simulink model "s_b2a4x1kf"  (R2018b)
settings: Solver=VariableStepDiscrete  StartTime=0.0  StopTime=100  RelTol=1e-3
undefined symbols (not defined in the file): fft_stages, n_bits_ants, n_bits_xengs
libraries: xbsIndex_r4 x20671, casper_library_misc x69, casper_library_scopes x15, casper_library_delays x8, xbsReplacements_r4 x6, xps_library x4
(part 152 of 212)

== system s_b2a4x1kf/sys0/xeng/baseline_tap1/dual_pol_cmac/cmac1 ==
  a+bi : Inport
  c+di : Inport  Port=2
  acc_in : Inport  Port=3
  sync : Inport  Port=4
  valid_in : Inport  Port=5
  Constant1 : xbsIndex_r4/Constant  const=0  gui_display_data_type=Fixed-point  arith_type=Unsigned  n_bits=bit_growth  bin_pt=0  preci_type=Single  exp_width=8  frac_width=24  explicit_period=on  period=1  equ=P=C  opselect=C  inp2=PCIN>>17  opr=+  inp1=P  carry=CIN  dbl_ovrd=off  block_type=constant
      settings: block_version=9.2.01
  Constant2 : xbsIndex_r4/Constant  const=0  gui_display_data_type=Fixed-point  arith_type=Unsigned  n_bits=1  bin_pt=0  preci_type=Single  exp_width=8  frac_width=24  explicit_period=off  period=1  equ=P=C  opselect=C  inp2=PCIN>>17  opr=+  inp1=P  carry=CIN  dbl_ovrd=off  block_type=constant
      settings: block_version=9.2.01
  Counter : xbsIndex_r4/Counter  cnt_type=Count Limited  cnt_to=acc_len - 1  operation=Up  start_count=0  cnt_by_val=1  arith_type=Unsigned  n_bits=bit_growth  bin_pt=0  load_pin=off  rst=on  en=off  explicit_period=off  period=1  use_behavioral_HDL=off  implementation=Fabric  use_rpm=on  dbl_ovrd=off  block_type=counter
      settings: xl_area=[0, 0, 0, 0, 0, 0, 0]  block_version=9.2.01
  Delay : xbsIndex_r4/Delay  rst=off  infoeditControl=Selection of Reset will increase slice count due to use of real FFs and instead of SRLs  en=off  latency=add_latency + mult_latency - 1  reg_retiming=on  dbl_ovrd=off  block_type=delay
      settings: xl_area=[0, 0, 0, 0, 0, 0, 0]  block_version=9.2.01
  Relational : xbsIndex_r4/Relational  mode=a=b  op_type=Bool  en=off  latency=1  dbl_ovrd=off  block_type=relational
      settings: xl_area=[0, 0, 0, 0, 0, 0, 0]  block_version=9.2.01
  Terminator : Terminator
  acc : Subsystem
  acc1 : Subsystem
  c_to_ri1 : Subsystem
  c_to_ri2 : Subsystem
  cmult* : Subsystem  AncestorBlock=casper_library_multipliers/cmult  mask(cmult){n_bits_a=8, bin_pt_a=7, n_bits_b=8, bin_pt_b=7, n_bits_ab=25, bin_pt_ab=14, quantization=Truncate, overflow=Wrap, in_latency=0, mult_latency=4, add_latency=3, conv_latency=0, conjugated=on, async=off, pipelined_enable=on, multiplier_implementation=embedded multiplier core}
      mask prompts: n_bits_a "Number of Bits 'a'"; bin_pt_a "Binary Point 'a'"; n_bits_b "Number of Bits 'b'"; bin_pt_b "Binary Point 'b'"; n_bits_ab "Number of Bits 'ab'"; bin_pt_ab "Binary Point 'ab'"; in_latency "Input latency"; mult_latency "Multiplier Latency"; add_latency "Adder Latency"; conv_latency "Convert latency"; conjugated "Conjugate"; async "asynchronous operation"; pipelined_enable "enable pipeline"; multiplier_implementation "Multiplier implementation"
      mask help:
      | Multiplies two complex numbers using 4 multipliers and 2 adders.
      | Conjugation is optional.
      mask init: same as s_b2a4x1kf/sys0/xeng/auto_tap/dual_pol_cmac/cmac/cmult*
      settings: AttributesFormatString=|
      | 8_7 * 8_7 ==> 25_14
      | Truncate, Wrap
      | Latency=0
      mask TypeOptions quantization: Truncate | Round  (unbiased: +/- Inf) | Round  (unbiased: Even Values)
      mask TypeOptions overflow: Wrap | Saturate | Flag as error
      mask TypeOptions multiplier_implementation: behavioral HDL | standard core | embedded multiplier core
  ri_to_c : Subsystem
  acc_out : Outport
  valid_out : Outport  Port=2
  wires:
  cmult*/1(ab) -> c_to_ri1/1(In1)
  valid_in/1 -> acc1/4(valid_in)
  acc1/2(valid_out) -> valid_out/1
  acc/2(valid_out) -> Terminator/1
  Constant2/1 -> acc/4(valid_in)
  Delay/1 -> Counter/1
  sync/1 -> Delay/1
  Constant1/1 -> Relational/2
  Counter/1 -> Relational/1
  Relational/1 -> acc1/1(rst), acc/1(rst)
  c_to_ri2/2(Out2) -> acc1/3(acc_in)
  ri_to_c/1(Out1) -> acc_out/1
  acc1/1(acc_out) -> ri_to_c/2(In2)
  acc_in/1 -> c_to_ri2/1(In1)
  c+di/1 -> cmult*/2(b)
  a+bi/1 -> cmult*/1(a)
  c_to_ri1/1(Out1) -> acc/2(din)  "auto_real"
  c_to_ri1/2(Out2) -> acc1/2(din)
  acc/1(acc_out) -> ri_to_c/1(In1)
  c_to_ri2/1(Out1) -> acc/3(acc_in)

== system s_b2a4x1kf/sys0/xeng/baseline_tap1/dual_pol_cmac/cmac2 ==
  a+bi : Inport
  c+di : Inport  Port=2
  acc_in : Inport  Port=3
  sync : Inport  Port=4
  valid_in : Inport  Port=5
  Constant1 : xbsIndex_r4/Constant  const=0  gui_display_data_type=Fixed-point  arith_type=Unsigned  n_bits=bit_growth  bin_pt=0  preci_type=Single  exp_width=8  frac_width=24  explicit_period=on  period=1  equ=P=C  opselect=C  inp2=PCIN>>17  opr=+  inp1=P  carry=CIN  dbl_ovrd=off  block_type=constant
      settings: block_version=9.2.01
  Constant2 : xbsIndex_r4/Constant  const=0  gui_display_data_type=Fixed-point  arith_type=Unsigned  n_bits=1  bin_pt=0  preci_type=Single  exp_width=8  frac_width=24  explicit_period=off  period=1  equ=P=C  opselect=C  inp2=PCIN>>17  opr=+  inp1=P  carry=CIN  dbl_ovrd=off  block_type=constant
      settings: block_version=9.2.01
  Counter : xbsIndex_r4/Counter  cnt_type=Count Limited  cnt_to=acc_len - 1  operation=Up  start_count=0  cnt_by_val=1  arith_type=Unsigned  n_bits=bit_growth  bin_pt=0  load_pin=off  rst=on  en=off  explicit_period=off  period=1  use_behavioral_HDL=off  implementation=Fabric  use_rpm=on  dbl_ovrd=off  block_type=counter
      settings: xl_area=[0, 0, 0, 0, 0, 0, 0]  block_version=9.2.01
  Delay : xbsIndex_r4/Delay  rst=off  infoeditControl=Selection of Reset will increase slice count due to use of real FFs and instead of SRLs  en=off  latency=add_latency + mult_latency - 1  reg_retiming=on  dbl_ovrd=off  block_type=delay
      settings: xl_area=[0, 0, 0, 0, 0, 0, 0]  block_version=9.2.01
  Relational : xbsIndex_r4/Relational  mode=a=b  op_type=Bool  en=off  latency=1  dbl_ovrd=off  block_type=relational
      settings: xl_area=[0, 0, 0, 0, 0, 0, 0]  block_version=9.2.01
  Terminator : Terminator
  acc : Subsystem
  acc1 : Subsystem
  c_to_ri1 : Subsystem
  c_to_ri2 : Subsystem
  cmult* : Subsystem  AncestorBlock=casper_library_multipliers/cmult  mask(cmult){n_bits_a=8, bin_pt_a=7, n_bits_b=8, bin_pt_b=7, n_bits_ab=25, bin_pt_ab=14, quantization=Truncate, overflow=Wrap, in_latency=0, mult_latency=4, add_latency=3, conv_latency=0, conjugated=on, async=off, pipelined_enable=on, multiplier_implementation=embedded multiplier core}
      mask prompts: n_bits_a "Number of Bits 'a'"; bin_pt_a "Binary Point 'a'"; n_bits_b "Number of Bits 'b'"; bin_pt_b "Binary Point 'b'"; n_bits_ab "Number of Bits 'ab'"; bin_pt_ab "Binary Point 'ab'"; in_latency "Input latency"; mult_latency "Multiplier Latency"; add_latency "Adder Latency"; conv_latency "Convert latency"; conjugated "Conjugate"; async "asynchronous operation"; pipelined_enable "enable pipeline"; multiplier_implementation "Multiplier implementation"
      mask help:
      | Multiplies two complex numbers using 4 multipliers and 2 adders.
      | Conjugation is optional.
      mask init: same as s_b2a4x1kf/sys0/xeng/auto_tap/dual_pol_cmac/cmac/cmult*
      settings: AttributesFormatString=|
      | 8_7 * 8_7 ==> 25_14
      | Truncate, Wrap
      | Latency=0
      mask TypeOptions quantization: Truncate | Round  (unbiased: +/- Inf) | Round  (unbiased: Even Values)
      mask TypeOptions overflow: Wrap | Saturate | Flag as error
      mask TypeOptions multiplier_implementation: behavioral HDL | standard core | embedded multiplier core
  ri_to_c : Subsystem
  acc_out : Outport
  valid_out : Outport  Port=2
  wires:
  cmult*/1(ab) -> c_to_ri1/1(In1)
  valid_in/1 -> acc1/4(valid_in)
  acc1/2(valid_out) -> valid_out/1
  acc/2(valid_out) -> Terminator/1
  Constant2/1 -> acc/4(valid_in)
  Delay/1 -> Counter/1
  sync/1 -> Delay/1
  Constant1/1 -> Relational/2
  Counter/1 -> Relational/1
  Relational/1 -> acc1/1(rst), acc/1(rst)
  c_to_ri2/2(Out2) -> acc1/3(acc_in)
  ri_to_c/1(Out1) -> acc_out/1
  acc1/1(acc_out) -> ri_to_c/2(In2)
  acc_in/1 -> c_to_ri2/1(In1)
  c+di/1 -> cmult*/2(b)
  a+bi/1 -> cmult*/1(a)
  c_to_ri1/1(Out1) -> acc/2(din)  "auto_real"
  c_to_ri1/2(Out2) -> acc1/2(din)
  acc/1(acc_out) -> ri_to_c/1(In1)
  c_to_ri2/1(Out1) -> acc/3(acc_in)

== system s_b2a4x1kf/sys0/xeng/baseline_tap1/dual_pol_cmac/cmac3 ==
  a+bi : Inport
  c+di : Inport  Port=2
  acc_in : Inport  Port=3
  sync : Inport  Port=4
  valid_in : Inport  Port=5
  Constant1 : xbsIndex_r4/Constant  const=0  gui_display_data_type=Fixed-point  arith_type=Unsigned  n_bits=bit_growth  bin_pt=0  preci_type=Single  exp_width=8  frac_width=24  explicit_period=on  period=1  equ=P=C  opselect=C  inp2=PCIN>>17  opr=+  inp1=P  carry=CIN  dbl_ovrd=off  block_type=constant
      settings: block_version=9.2.01
  Constant2 : xbsIndex_r4/Constant  const=0  gui_display_data_type=Fixed-point  arith_type=Unsigned  n_bits=1  bin_pt=0  preci_type=Single  exp_width=8  frac_width=24  explicit_period=off  period=1  equ=P=C  opselect=C  inp2=PCIN>>17  opr=+  inp1=P  carry=CIN  dbl_ovrd=off  block_type=constant
      settings: block_version=9.2.01
  Counter : xbsIndex_r4/Counter  cnt_type=Count Limited  cnt_to=acc_len - 1  operation=Up  start_count=0  cnt_by_val=1  arith_type=Unsigned  n_bits=bit_growth  bin_pt=0  load_pin=off  rst=on  en=off  explicit_period=off  period=1  use_behavioral_HDL=off  implementation=Fabric  use_rpm=on  dbl_ovrd=off  block_type=counter
      settings: xl_area=[0, 0, 0, 0, 0, 0, 0]  block_version=9.2.01
  Delay : xbsIndex_r4/Delay  rst=off  infoeditControl=Selection of Reset will increase slice count due to use of real FFs and instead of SRLs  en=off  latency=add_latency + mult_latency - 1  reg_retiming=on  dbl_ovrd=off  block_type=delay
      settings: xl_area=[0, 0, 0, 0, 0, 0, 0]  block_version=9.2.01
  Relational : xbsIndex_r4/Relational  mode=a=b  op_type=Bool  en=off  latency=1  dbl_ovrd=off  block_type=relational
      settings: xl_area=[0, 0, 0, 0, 0, 0, 0]  block_version=9.2.01
  Terminator : Terminator
  acc : Subsystem
  acc1 : Subsystem
  c_to_ri1 : Subsystem
  c_to_ri2 : Subsystem
  cmult* : Subsystem  AncestorBlock=casper_library_multipliers/cmult  mask(cmult){n_bits_a=8, bin_pt_a=7, n_bits_b=8, bin_pt_b=7, n_bits_ab=25, bin_pt_ab=14, quantization=Truncate, overflow=Wrap, in_latency=0, mult_latency=4, add_latency=3, conv_latency=0, conjugated=on, async=off, pipelined_enable=on, multiplier_implementation=embedded multiplier core}
      mask prompts: n_bits_a "Number of Bits 'a'"; bin_pt_a "Binary Point 'a'"; n_bits_b "Number of Bits 'b'"; bin_pt_b "Binary Point 'b'"; n_bits_ab "Number of Bits 'ab'"; bin_pt_ab "Binary Point 'ab'"; in_latency "Input latency"; mult_latency "Multiplier Latency"; add_latency "Adder Latency"; conv_latency "Convert latency"; conjugated "Conjugate"; async "asynchronous operation"; pipelined_enable "enable pipeline"; multiplier_implementation "Multiplier implementation"
      mask help:
      | Multiplies two complex numbers using 4 multipliers and 2 adders.
      | Conjugation is optional.
      mask init: same as s_b2a4x1kf/sys0/xeng/auto_tap/dual_pol_cmac/cmac/cmult*
      settings: AttributesFormatString=|
      | 8_7 * 8_7 ==> 25_14
      | Truncate, Wrap
      | Latency=0
      mask TypeOptions quantization: Truncate | Round  (unbiased: +/- Inf) | Round  (unbiased: Even Values)
      mask TypeOptions overflow: Wrap | Saturate | Flag as error
      mask TypeOptions multiplier_implementation: behavioral HDL | standard core | embedded multiplier core
  ri_to_c : Subsystem
  acc_out : Outport
  valid_out : Outport  Port=2
  wires:
  cmult*/1(ab) -> c_to_ri1/1(In1)
  valid_in/1 -> acc1/4(valid_in)
  acc1/2(valid_out) -> valid_out/1
  acc/2(valid_out) -> Terminator/1
  Constant2/1 -> acc/4(valid_in)
  Delay/1 -> Counter/1
  sync/1 -> Delay/1
  Constant1/1 -> Relational/2
  Counter/1 -> Relational/1
  Relational/1 -> acc1/1(rst), acc/1(rst)
  c_to_ri2/2(Out2) -> acc1/3(acc_in)
  ri_to_c/1(Out1) -> acc_out/1
  acc1/1(acc_out) -> ri_to_c/2(In2)
  acc_in/1 -> c_to_ri2/1(In1)
  c+di/1 -> cmult*/2(b)
  a+bi/1 -> cmult*/1(a)
  c_to_ri1/1(Out1) -> acc/2(din)  "auto_real"
  c_to_ri1/2(Out2) -> acc1/2(din)
  acc/1(acc_out) -> ri_to_c/1(In1)
  c_to_ri2/1(Out1) -> acc/3(acc_in)

== system s_b2a4x1kf/sys0/xeng/xeng_descramble/write_ctrl/negedge_delay ==
  in : Inport
  Constant5 : xbsIndex_r4/Constant  const=pulse_len-2  gui_display_data_type=Fixed-point  arith_type=Unsigned  n_bits=bits  bin_pt=0  preci_type=Single  exp_width=8  frac_width=24  explicit_period=off  period=1  equ=P=C  opselect=C  inp2=PCIN>>17  opr=+  inp1=P  carry=CIN  dbl_ovrd=off  block_type=constant
      settings: block_version=9.1.01
  Counter3 : xbsIndex_r4/Counter  cnt_type=Free Running  cnt_to=1023  operation=Up  start_count=0  cnt_by_val=1  arith_type=Unsigned  n_bits=bits  bin_pt=0  load_pin=off  rst=on  en=on  explicit_period=on  period=1  use_behavioral_HDL=off  implementation=Fabric  use_rpm=on  dbl_ovrd=off  block_type=counter
      settings: xl_area=[0, 0, 0, 0, 0, 0, 0]  block_version=9.1.01
  Delay : xbsIndex_r4/Delay  rst=off  infoeditControl=Selection of Reset will increase slice count due to use of real FFs and instead of SRLs  en=off  latency=1  reg_retiming=on  dbl_ovrd=off  block_type=delay
  Logical : xbsIndex_r4/Logical  logical_function=OR  inputs=3  en=off  latency=0  precision=Full  arith_type=Unsigned  n_bits=16  bin_pt=0  align_bp=on  dbl_ovrd=off  block_type=logical
  Relational5 : xbsIndex_r4/Relational  mode=a<=b  op_type=Bool  en=off  latency=0  dbl_ovrd=off  block_type=relational
      settings: xl_area=[0, 0, 0, 0, 0, 0, 0]  block_version=9.1.01
  negedge : Subsystem  AncestorBlock=casper_library_misc/edge_detect  mask(edge_detect){edge=Falling, polarity=Active High, x_in=[0 0.08 0.08 0.16 0.16 0.24 0.24 0.32 0.32 0.4], y_in=[-1 -1  1  1  1  1  1  1  1  1], x_out=[0.6 0.68 0.68 0.76 0.76 0.84 0.84 0.92 0.92 1], y_out=[-1 -1  1  1 -1 -1 -1 -1 -1 -1]}
      mask prompts: edge "Edge Type"; polarity "Output Polarity"; x_in "Input X Positions"; y_in "Input Y Positions"; x_out "Output X Positions"; y_out "Output Y Positions"
      mask help: Output is active for one-cycle after each edge of the specified type (i.e. rising, falling or both).
      mask init: same as s_b2a4x1kf/edge_detect
      settings: AttributesFormatString=|
      | falling edges
      | active high
      mask Help: Output is active for one-cycle after each edge of the specified type (i.e. rising, falling, or both).  Latency is zero.
      mask TypeOptions edge: Rising | Falling | Both
      mask TypeOptions polarity: Active High | Active Low
      mask Display:
      | plot(x_in_num,0.5+y_in_num*0.2);
      | plot(x_out_num,0.5+y_out_num*0.2);
  out : Outport
  wires:
  Delay/1 -> Logical/2
  Logical/1 -> out/1
  Counter3/1 -> Relational5/1
  Constant5/1 -> Relational5/2
  Relational5/1 -> Logical/3, Counter3/2
  in/1 -> Logical/1, Delay/1, negedge/1(in)
  negedge/1(out) -> Counter3/1

== system s_b2a4x1kf/sys1/bf/fbf/apply_beam_weights/bus_convert ==
  din : Inport
  misci : Inport  Port=2
  bussify : Subsystem  mask(bus_create){inputNum=4}
      mask prompts: inputNum "Number of inputs:"
      mask init:
      | bus_create_init(gcb,...
      |     'inputNum', inputNum);
  conv1 : Subsystem  mask(convert){bin_pt_in=16, n_bits_out=25, bin_pt_out=16, quantization=Truncate, overflow=Wrap, csp_latency=0}
      mask prompts: bin_pt_in "Binary Point In"; n_bits_out "Bit Width Out"; bin_pt_out "Binary Point Out"; csp_latency "Latency"
      mask help:
      | Convert input value to the specified bit width and precision.
      |
      | Does not support upscaling number of fractional bits (eg 8_5 to 8_4 is ok, but not 8_4 to 8_5).
      mask init: same as s_b2a4x1kf/sys0/31->32/conv1
      settings: AttributesFormatString=|
      | N_16 ==> 25_16
      | truncate, wrap
      | latency = 0
      mask Help:
      | <pre>
      | Description::
      | 
      | Outputs converted version of the input.
      | 
      | Mask Parameters::
      | 
      | Binary Point In (bin_pt_in): Specifies the binary point location in the input.
      | 
      | Bit Width Out (n_bits_out): Specifies the width of the output.
      | 
      | Binary Point Out (bin_pt_out): Specifies the binary point location in the output.
      | 
      | Quantization (quantization): Specifies quantization handling.
      | 
      | Overflow (overflow): Specifies overflow handling.
      | 
      | Latency (latency): Specifies the latency of the underlying adder block, which is the overall
      | latency of this block as well.
      | </pre>
      mask TypeOptions quantization: Truncate | Round  (unbiased: +/- Inf) | Round  (unbiased: Even Values) | Round  (unbiased: Zero) | Round  (unbiased: Odd Values) | Round  (biased: Up) | Round  (biased: Down)
      mask TypeOptions overflow: Wrap | Saturate | Error
  conv2 : Subsystem  mask(convert){bin_pt_in=16, n_bits_out=25, bin_pt_out=16, quantization=Truncate, overflow=Wrap, csp_latency=0}
      mask prompts: bin_pt_in "Binary Point In"; n_bits_out "Bit Width Out"; bin_pt_out "Binary Point Out"; csp_latency "Latency"
      mask help:
      | Convert input value to the specified bit width and precision.
      |
      | Does not support upscaling number of fractional bits (eg 8_5 to 8_4 is ok, but not 8_4 to 8_5).
      mask init: same as s_b2a4x1kf/sys0/31->32/conv1
      settings: AttributesFormatString=|
      | N_16 ==> 25_16
      | truncate, wrap
      | latency = 0
      mask Help:
      | <pre>
      | Description::
      | 
      | Outputs converted version of the input.
      | 
      | Mask Parameters::
      | 
      | Binary Point In (bin_pt_in): Specifies the binary point location in the input.
      | 
      | Bit Width Out (n_bits_out): Specifies the width of the output.
      | 
      | Binary Point Out (bin_pt_out): Specifies the binary point location in the output.
      | 
      | Quantization (quantization): Specifies quantization handling.
      | 
      | Overflow (overflow): Specifies overflow handling.
      | 
      | Latency (latency): Specifies the latency of the underlying adder block, which is the overall
      | latency of this block as well.
      | </pre>
      mask TypeOptions quantization: Truncate | Round  (unbiased: +/- Inf) | Round  (unbiased: Even Values) | Round  (unbiased: Zero) | Round  (unbiased: Odd Values) | Round  (biased: Up) | Round  (biased: Down)
      mask TypeOptions overflow: Wrap | Saturate | Error
  conv3 : Subsystem  mask(convert){bin_pt_in=16, n_bits_out=25, bin_pt_out=16, quantization=Truncate, overflow=Wrap, csp_latency=0}
      mask prompts: bin_pt_in "Binary Point In"; n_bits_out "Bit Width Out"; bin_pt_out "Binary Point Out"; csp_latency "Latency"
      mask help:
      | Convert input value to the specified bit width and precision.
      |
      | Does not support upscaling number of fractional bits (eg 8_5 to 8_4 is ok, but not 8_4 to 8_5).
      mask init: same as s_b2a4x1kf/sys0/31->32/conv1
      settings: AttributesFormatString=|
      | N_16 ==> 25_16
      | truncate, wrap
      | latency = 0
      mask Help:
      | <pre>
      | Description::
      | 
      | Outputs converted version of the input.
      | 
      | Mask Parameters::
      | 
      | Binary Point In (bin_pt_in): Specifies the binary point location in the input.
      | 
      | Bit Width Out (n_bits_out): Specifies the width of the output.
      | 
      | Binary Point Out (bin_pt_out): Specifies the binary point location in the output.
      | 
      | Quantization (quantization): Specifies quantization handling.
      | 
      | Overflow (overflow): Specifies overflow handling.
      | 
      | Latency (latency): Specifies the latency of the underlying adder block, which is the overall
      | latency of this block as well.
      | </pre>
      mask TypeOptions quantization: Truncate | Round  (unbiased: +/- Inf) | Round  (unbiased: Even Values) | Round  (unbiased: Zero) | Round  (unbiased: Odd Values) | Round  (biased: Up) | Round  (biased: Down)
      mask TypeOptions overflow: Wrap | Saturate | Error
  conv4 : Subsystem  mask(convert){bin_pt_in=16, n_bits_out=25, bin_pt_out=16, quantization=Truncate, overflow=Wrap, csp_latency=0}
      mask prompts: bin_pt_in "Binary Point In"; n_bits_out "Bit Width Out"; bin_pt_out "Binary Point Out"; csp_latency "Latency"
      mask help:
      | Convert input value to the specified bit width and precision.
      |
      | Does not support upscaling number of fractional bits (eg 8_5 to 8_4 is ok, but not 8_4 to 8_5).
      mask init: same as s_b2a4x1kf/sys0/31->32/conv1
      settings: AttributesFormatString=|
      | N_16 ==> 25_16
      | truncate, wrap
      | latency = 0
      mask Help:
      | <pre>
      | Description::
      | 
      | Outputs converted version of the input.
      | 
      | Mask Parameters::
      | 
      | Binary Point In (bin_pt_in): Specifies the binary point location in the input.
      | 
      | Bit Width Out (n_bits_out): Specifies the width of the output.
      | 
      | Binary Point Out (bin_pt_out): Specifies the binary point location in the output.
      | 
      | Quantization (quantization): Specifies quantization handling.
      | 
      | Overflow (overflow): Specifies overflow handling.
      | 
      | Latency (latency): Specifies the latency of the underlying adder block, which is the overall
      | latency of this block as well.
      | </pre>
      mask TypeOptions quantization: Truncate | Round  (unbiased: +/- Inf) | Round  (unbiased: Even Values) | Round  (unbiased: Zero) | Round  (unbiased: Odd Values) | Round  (biased: Up) | Round  (biased: Down)
      mask TypeOptions overflow: Wrap | Saturate | Error
  debus : Subsystem  mask(bus_expand){mode=divisions of arbitrary size, outputNum=1, outputWidth=[25 25 25 25], outputBinaryPt=[16 16 16 16], outputArithmeticType=[1 1 1 1], show_format=on, outputToWorkspace=off, variablePrefix=, outputToModelAsWell=on}
      mask prompts: outputNum "Number of outputs:"; outputWidth "Output width [msb ... lsb]:"; outputBinaryPt "Output binary point position [msb ... lsb]:"; outputArithmeticType "Output arithmetic type (ufix=0, fix=1, bool=2) [msb ... lsb]:"; show_format "Print format string?"; outputToWorkspace "Output to workspace?"; variablePrefix "Variable name prefix:"; outputToModelAsWell "Output to model as well?"
      mask help:
      | Expands a 'bus' made using a bus_create or Xilinx
      | concat block.
      | The input will be divided into the specified number
      | of outputs with the specified arithmetic types.
      | Divisions are made from most significant bit.
      mask init: same as s_b2a4x1kf/bus_expand
      settings: AttributesFormatString=4 outputs: f25.16,f25.16,f25.16,f25.16,
      mask TypeOptions mode: divisions of equal size | divisions of arbitrary size
      mask Callback mode: bus_expand_callback();
      mask Callback outputWidth: bus_expand_callback();
      mask Callback outputToWorkspace: bus_expand_callback();
  dmisc : xbsIndex_r4/Delay  rst=off  infoeditControl=Selection of Reset will increase slice count due to use of real FFs and instead of SRLs  en=off  latency=csp_latency  reg_retiming=on  dbl_ovrd=off  block_type=delay
  dout : Outport
  misco : Outport  Port=2
  wires:
  din/1 -> debus/1(bus_in)
  debus/1(msb_out4) -> conv1/1(in)
  debus/2(out3) -> conv2/1(in)
  debus/3(out2) -> conv3/1(in)
  debus/4(lsb_out1) -> conv4/1(in)
  misci/1 -> dmisc/1
  conv1/1(out) -> bussify/1(in1)
  conv2/1(out) -> bussify/2(in2)
  conv3/1(out) -> bussify/3(in3)
  conv4/1(out) -> bussify/4(in4)
  bussify/1(bus_out) -> dout/1
  dmisc/1 -> misco/1

== system s_b2a4x1kf/sys1/bf/fbf/apply_beam_weights/bus_mult ==
  a : Inport
  b : Inport  Port=2
  misci : Inport  Port=3
  a*b_bussify : Subsystem  mask(bus_create){inputNum=4}
      mask prompts: inputNum "Number of inputs:"
      mask init:
      | bus_create_init(gcb,...
      |     'inputNum', inputNum);
  a_debus : Subsystem  mask(bus_expand){mode=divisions of arbitrary size, outputNum=1, outputWidth=[8 8 8 8], outputBinaryPt=[7 7 7 7], outputArithmeticType=[1 1 1 1], show_format=on, outputToWorkspace=off, variablePrefix=, outputToModelAsWell=on}
      mask prompts: outputNum "Number of outputs:"; outputWidth "Output width [msb ... lsb]:"; outputBinaryPt "Output binary point position [msb ... lsb]:"; outputArithmeticType "Output arithmetic type (ufix=0, fix=1, bool=2) [msb ... lsb]:"; show_format "Print format string?"; outputToWorkspace "Output to workspace?"; variablePrefix "Variable name prefix:"; outputToModelAsWell "Output to model as well?"
      mask help:
      | Expands a 'bus' made using a bus_create or Xilinx
      | concat block.
      | The input will be divided into the specified number
      | of outputs with the specified arithmetic types.
      | Divisions are made from most significant bit.
      mask init: same as s_b2a4x1kf/bus_expand
      settings: AttributesFormatString=4 outputs: f8.7,f8.7,f8.7,f8.7,
      mask TypeOptions mode: divisions of equal size | divisions of arbitrary size
      mask Callback mode: bus_expand_callback();
      mask Callback outputWidth: bus_expand_callback();
      mask Callback outputToWorkspace: bus_expand_callback();
  b_debus : Subsystem  mask(bus_expand){mode=divisions of arbitrary size, outputNum=1, outputWidth=[16 16], outputBinaryPt=[9 9], outputArithmeticType=[1 1], show_format=on, outputToWorkspace=off, variablePrefix=, outputToModelAsWell=on}
      mask prompts: outputNum "Number of outputs:"; outputWidth "Output width [msb ... lsb]:"; outputBinaryPt "Output binary point position [msb ... lsb]:"; outputArithmeticType "Output arithmetic type (ufix=0, fix=1, bool=2) [msb ... lsb]:"; show_format "Print format string?"; outputToWorkspace "Output to workspace?"; variablePrefix "Variable name prefix:"; outputToModelAsWell "Output to model as well?"
      mask help:
      | Expands a 'bus' made using a bus_create or Xilinx
      | concat block.
      | The input will be divided into the specified number
      | of outputs with the specified arithmetic types.
      | Divisions are made from most significant bit.
      mask init: same as s_b2a4x1kf/bus_expand
      settings: AttributesFormatString=2 outputs: f16.9,f16.9,
      mask TypeOptions mode: divisions of equal size | divisions of arbitrary size
      mask Callback mode: bus_expand_callback();
      mask Callback outputWidth: bus_expand_callback();
      mask Callback outputToWorkspace: bus_expand_callback();
  dmisc : xbsIndex_r4/Delay  rst=off  infoeditControl=Selection of Reset will increase slice count due to use of real FFs and instead of SRLs  en=off  latency=mult_latency+fan_latency  reg_retiming=on  dbl_ovrd=off  block_type=delay
      settings: infoedit=Hardware notes: A delay line is a chain, each link of which is an SRL16 or SRL32 followed by a flip-flop.
  mult{1..4} (4 alike) : xbsIndex_r4/Mult  precision=User Defined  arith_type="Signed  (2's comp)"  n_bits=25  bin_pt=16  quantization=Truncate  overflow=Wrap  en=off  latency=mult_latency  use_behavioral_HDL=off  opt=Speed  use_embedded=on  optimum_pipeline=off  pipeline=on  dbl_ovrd=off  use_rpm=on  placement_style=Triangular  block_type=mult
  repa : Subsystem  Tag=cmac_delinked  mask(bus_replicate){replication=1, csp_latency=1, misc=off, implementation=core}
      mask prompts: replication "replication factor"; csp_latency "latency"; misc "misc support"; implementation "delay implementation"
      mask help: Output bus formed by replicating input bus a number of times
      mask init:
      | bus_replicate_init(gcb, ...
      |     'replication', replication, ...
      |     'csp_latency', csp_latency, ...
      |     'implementation', implementation, ...
      |     'misc', misc);
      mask TypeOptions implementation: core | behavioral
  repb : Subsystem  mask(bus_replicate){replication=1, csp_latency=1, misc=off, implementation=core}
      mask prompts: replication "replication factor"; csp_latency "latency"; misc "misc support"; implementation "delay implementation"
      mask help: Output bus formed by replicating input bus a number of times
      mask init:
      | bus_replicate_init(gcb, ...
      |     'replication', replication, ...
      |     'csp_latency', csp_latency, ...
      |     'implementation', implementation, ...
      |     'misc', misc);
      mask TypeOptions implementation: core | behavioral
  a*b : Outport
  misco : Outport  Port=2
  wires:
  a/1 -> repa/1(in)
  b/1 -> repb/1(in)
  repa/1(out) -> a_debus/1(bus_in)
  repb/1(out) -> b_debus/1(bus_in)
  a_debus/1(msb_out4) -> mult1/1
  b_debus/1(msb_out2) -> mult1/2, mult2/2
  a_debus/2(out3) -> mult2/1
  a_debus/3(out2) -> mult3/1
  b_debus/2(lsb_out1) -> mult3/2, mult4/2
  a_debus/4(lsb_out1) -> mult4/1
  misci/1 -> dmisc/1
  mult1/1 -> a*b_bussify/1(in1)
  mult2/1 -> a*b_bussify/2(in2)
  mult3/1 -> a*b_bussify/3(in3)
  mult4/1 -> a*b_bussify/4(in4)
  a*b_bussify/1(bus_out) -> a*b/1
  dmisc/1 -> misco/1

== system s_b2a4x1kf/sys1/bf/fbf/apply_beam_weights/munge_in ==
  din : Inport
  join : Subsystem  mask(bus_create){inputNum=2}
      mask prompts: inputNum "Number of inputs:"
      mask init:
      | bus_create_init(gcb,...
      |     'inputNum', inputNum);
  reinterpret : xbsIndex_r4/Reinterpret  force_arith_type=on  arith_type=Unsigned  force_bin_pt=on  bin_pt=0  block_type=reinterpret
  reinterpret_out : xbsIndex_r4/Reinterpret  force_arith_type=on  arith_type=Unsigned  force_bin_pt=on  bin_pt=0  block_type=reinterpret
  split : Subsystem  mask(bus_expand){mode=divisions of arbitrary size, outputNum=1, outputWidth=[16 16], outputBinaryPt=[0 0], outputArithmeticType=[0 0], show_format=off, outputToWorkspace=off, variablePrefix=out, outputToModelAsWell=on}
      mask prompts: outputNum "Number of outputs:"; outputWidth "Output width [msb ... lsb]:"; outputBinaryPt "Output binary point position [msb ... lsb]:"; outputArithmeticType "Output arithmetic type (ufix=0, fix=1, bool=2) [msb ... lsb]:"; show_format "Print format string?"; outputToWorkspace "Output to workspace?"; variablePrefix "Variable name prefix:"; outputToModelAsWell "Output to model as well?"
      mask help:
      | Expands a 'bus' made using a bus_create or Xilinx
      | concat block.
      | The input will be divided into the specified number
      | of outputs with the specified arithmetic types.
      | Divisions are made from most significant bit.
      mask init: same as s_b2a4x1kf/bus_expand
      settings: AttributesFormatString=2 outputs
      mask TypeOptions mode: divisions of equal size | divisions of arbitrary size
      mask Callback mode: bus_expand_callback();
      mask Callback outputWidth: bus_expand_callback();
      mask Callback outputToWorkspace: bus_expand_callback();
  dout : Outport
  wires:
  reinterpret_out/1 -> dout/1
  din/1 -> reinterpret/1
  reinterpret/1 -> split/1(bus_in)
  join/1(bus_out) -> reinterpret_out/1
  split/2(lsb_out1) -> join/1(in1)
  split/1(msb_out2) -> join/2(in2)

== system s_b2a4x1kf/sys1/bf/fbf/apply_beam_weights/munge_out ==
  din : Inport
  join : Subsystem  mask(bus_create){inputNum=2}
      mask prompts: inputNum "Number of inputs:"
      mask init:
      | bus_create_init(gcb,...
      |     'inputNum', inputNum);
  reinterpret : xbsIndex_r4/Reinterpret  force_arith_type=on  arith_type=Unsigned  force_bin_pt=on  bin_pt=0  block_type=reinterpret
  reinterpret_out : xbsIndex_r4/Reinterpret  force_arith_type=on  arith_type=Unsigned  force_bin_pt=on  bin_pt=0  block_type=reinterpret
  split : Subsystem  mask(bus_expand){mode=divisions of arbitrary size, outputNum=1, outputWidth=[50 50], outputBinaryPt=[0 0], outputArithmeticType=[0 0], show_format=off, outputToWorkspace=off, variablePrefix=out, outputToModelAsWell=on}
      mask prompts: outputNum "Number of outputs:"; outputWidth "Output width [msb ... lsb]:"; outputBinaryPt "Output binary point position [msb ... lsb]:"; outputArithmeticType "Output arithmetic type (ufix=0, fix=1, bool=2) [msb ... lsb]:"; show_format "Print format string?"; outputToWorkspace "Output to workspace?"; variablePrefix "Variable name prefix:"; outputToModelAsWell "Output to model as well?"
      mask help:
      | Expands a 'bus' made using a bus_create or Xilinx
      | concat block.
      | The input will be divided into the specified number
      | of outputs with the specified arithmetic types.
      | Divisions are made from most significant bit.
      mask init: same as s_b2a4x1kf/bus_expand
      settings: AttributesFormatString=2 outputs
      mask TypeOptions mode: divisions of equal size | divisions of arbitrary size
      mask Callback mode: bus_expand_callback();
      mask Callback outputWidth: bus_expand_callback();
      mask Callback outputToWorkspace: bus_expand_callback();
  dout : Outport
  wires:
  reinterpret_out/1 -> dout/1
  din/1 -> reinterpret/1
  reinterpret/1 -> split/1(bus_in)
  join/1(bus_out) -> reinterpret_out/1
  split/2(lsb_out1) -> join/1(in1)
  split/1(msb_out2) -> join/2(in2)

== system s_b2a4x1kf/sys1/bf/fbf/combine/acc ==
  note: accumulated data is
      | stored here
  note: generate 0s to
      | write back when
      | dumping in
      | preparation for
      | next integration
  note: add the stored value
      | to the incoming value
      | if data valid
  note: generate
      | correct address
      | whether data is
      | valid  or not
  note: enable addition
      | of input value
  note: indicates end of
      | accumulation,
      | may be high even
      | if data not valid
  synci : Inport
  dat : Inport  Port=2
  en : Inport  Port=3
  dvalid : Inport  Port=4
  dump : Inport  Port=5
  misc_in : Inport  Port=6
  Concat : xbsIndex_r4/Concat  num_inputs=4  dbl_ovrd=off  block_type=concat
  Concat1 : xbsIndex_r4/Concat  num_inputs=2  dbl_ovrd=off  block_type=concat
  Constant1 : xbsIndex_r4/Constant  const=0  gui_display_data_type=Fixed-point  arith_type=Unsigned  n_bits=n_bits_accum*2*2^stream_bits  bin_pt=0  preci_type=Single  exp_width=8  frac_width=24  explicit_period=on  period=1  equ=P=C  opselect=C  inp2=PCIN>>17  opr=+  inp1=P  carry=CIN  dbl_ovrd=off  block_type=constant
      settings: block_version=11.4
  Constant2 : xbsIndex_r4/Constant  const=0  gui_display_data_type=Fixed-point  arith_type=Boolean  n_bits=1  bin_pt=0  preci_type=Single  exp_width=8  frac_width=24  explicit_period=on  period=1  equ=P=C  opselect=C  inp2=PCIN>>17  opr=+  inp1=P  carry=CIN  dbl_ovrd=off  block_type=constant
      settings: block_version=11.4
  Delay{,2..5,8,11,17..18} (9 alike) : xbsIndex_r4/Delay  rst=off  infoeditControl=Selection of Reset will increase slice count due to use of real FFs and instead of SRLs  en=off  latency=bram_latency  reg_retiming=off  dbl_ovrd=off  block_type=delay
      Delay settings: infoedit=Hardware notes: A delay line is a chain, each link of which is an SRL16 or SRL32 followed by a flip-flop.  block_version=11.4
      Delay11 settings: infoedit=Hardware notes: A delay line is a chain, each link of which is an SRL16 or SRL32 followed by a flip-flop.  block_version=11.4
      Delay17 settings: infoedit=Hardware notes: A delay line is a chain, each link of which is an SRL16 or SRL32 followed by a flip-flop.  block_version=11.4
      Delay18 settings: infoedit=Hardware notes: A delay line is a chain, each link of which is an SRL16 or SRL32 followed by a flip-flop.  block_version=11.4
      Delay2 settings: block_version=11.4
      Delay3 settings: block_version=11.4
      Delay4 settings: block_version=11.4
      Delay5 settings: block_version=11.4
      Delay8 settings: block_version=11.4
  Delay{1,6..7,9,13..16,19,21..23} (12 alike) : xbsIndex_r4/Delay  rst=off  infoeditControl=Selection of Reset will increase slice count due to use of real FFs and instead of SRLs  en=off  latency=1  reg_retiming=off  dbl_ovrd=off  block_type=delay
      Delay1 settings: block_version=11.4
      Delay13 settings: infoedit=Hardware notes: A delay line is a chain, each link of which is an SRL16 or SRL32 followed by a flip-flop.  block_version=11.4
      Delay14 settings: infoedit=Hardware notes: A delay line is a chain, each link of which is an SRL16 or SRL32 followed by a flip-flop.  block_version=11.4
      Delay15 settings: infoedit=Hardware notes: A delay line is a chain, each link of which is an SRL16 or SRL32 followed by a flip-flop.  block_version=11.4
      Delay16 settings: infoedit=Hardware notes: A delay line is a chain, each link of which is an SRL16 or SRL32 followed by a flip-flop.  block_version=11.4
      Delay19 settings: block_version=11.4
      Delay21 settings: block_version=11.4
      Delay22 settings: block_version=11.4
      Delay23 settings: block_version=11.4
      Delay6 settings: block_version=11.4
      Delay7 settings: block_version=11.4
      Delay9 settings: block_version=11.4
  Delay10 : xbsIndex_r4/Delay  rst=off  infoeditControl=Selection of Reset will increase slice count due to use of real FFs and instead of SRLs  en=on  latency=1  reg_retiming=off  dbl_ovrd=off  block_type=delay
      settings: infoedit=Hardware notes: A delay line is a chain, each link of which is an SRL16 or SRL32 followed by a flip-flop.  block_version=11.4
  Delay12 : xbsIndex_r4/Delay  rst=off  infoeditControl=Selection of Reset will increase slice count due to use of real FFs and instead of SRLs  en=on  latency=1  reg_retiming=off  dbl_ovrd=off  block_type=delay
      settings: infoedit=Hardware notes: A delay line is a chain, each link of which is an SRL16 or SRL32 followed by a flip-flop.  block_version=11.4
  Delay20 : xbsIndex_r4/Delay  rst=off  infoeditControl=Selection of Reset will increase slice count due to use of real FFs and instead of SRLs  en=on  latency=1  reg_retiming=off  dbl_ovrd=off  block_type=delay
      settings: infoedit=Hardware notes: A delay line is a chain, each link of which is an SRL16 or SRL32 followed by a flip-flop.  block_version=11.4
  Gateway Out{,1..12} (13 alike) : xbsIndex_r4/Gateway Out  inherit_from_input=off  hdl_port=off  rows=1  columns=1  UseAsDAC=off  DACChannel='1'  interface=None  automatic_assignment=on  address_offset=hex2dec('00')  intf_name=''  intf_description=''  timing_constraint=None  locs_specified=off  LOCs={}  io_standard={}  block_type=gatewayout
      settings: infoedit="Gateway out block.  Converts Xilinx fixed point inputs into ouputs of type Simulink integer, double, or fixed point.<br><br>Hardware notes:  In hardware these blocks become top level output ports or are discarded, depending on how they are configured."  block_version=11.4
  Inverter : xbsIndex_r4/Inverter  en=off  latency=0  dbl_ovrd=off  block_type=inv
      settings: block_version=11.4
  Logical : xbsIndex_r4/Logical  logical_function=AND  inputs=2  en=off  latency=1  precision=Full  arith_type=Unsigned  n_bits=16  bin_pt=0  align_bp=on  dbl_ovrd=off  block_type=logical
      settings: block_version=11.4
  Register : xbsIndex_r4/Register  init=0  rst=on  en=off  dbl_ovrd=off  block_type=register
      settings: block_version=11.4
  Scope : Scope  NumInputPorts=5
  Scope1 : Scope  NumInputPorts=8
  Terminator : Terminator
  acc : xbsIndex_r4/Dual Port RAM  depth=2^stack_bits  initVector=zeros(2^stack_bits,1)  distributed_mem=Block RAM  init_a=0  init_b=0  rst_a=off  rst_b=off  en_a=off  en_b=off  latency=bram_latency  write_mode_A=Read Before Write  write_mode_B=Read Before Write  optimize=Area  dbl_ovrd=off  block_type=dpram
      settings: block_version=11.4
  bus_add : Subsystem  Tag=cmac_delinked  mask(bus_addsub){opmode=0, n_bits_a=repmat(n_bits_in, 1, 2^stream_bits), bin_pt_a=bin_pt_in, type_a=1, n_bits_b=repmat(n_bits_accum, 1, 2^stream_bits), bin_pt_b=bin_pt_in, type_b=1, cmplx=on, misc=on, async=off, floating_point=off, float_type=single, exp_width=6, frac_width=19, n_bits_out=n_bits_accum, bin_pt_out=bin_pt_in, type_out=1, quantization=0, overflow=0, add_implementation=behavioral HDL, csp_latency=add_latency, pipeline_en=off, pipeline_latency=0}
      mask prompts: opmode "mode (Addition=0, Subtraction=1)"; n_bits_a "a input bit widths"; bin_pt_a "a input binary points"; type_a "a input type (Unsigned=0, Signed=1)"; n_bits_b "b input bit widths"; bin_pt_b "b input binary points"; type_b "b input type (Unsigned=0, Signed=1)"; cmplx "complex"; misc "misc support"; async "asynchronous operation"; floating_point "floating point"; exp_width "exponent width"; frac_width "fraction width"; n_bits_out "output bit widths"; bin_pt_out "output binary points"; type_out "output type (Unsigned=0, Signed=1)"; quantization "quantization strategy (Truncate=0, Round  (unbiased: +/- Inf)=1)"; overflow "overflow strategy (Wrap=0, Saturate=1, Flag as error=2)"; add_implementation "adder implementation"; csp_latency "latency"; pipeline_en "pipeline enable"; pipeline_latency "pipeline latency"
      mask help: Add/subtract components of two busses
      mask init: same as s_b2a4x1kf/bus_addsub
      mask Callback floating_point:
      | onoff = get_param(gcb, 'floating_point');
      | if strcmp(onoff,'on')
      |     enable_fixpt = 'off'
      |     set_param_state(gcb, 'float_type', 'on')
      | 
      |     f_type = get_param(gcb, 'float_type')
      |     if strcmp(f_type,'custom')
      |         set_param_state(gcb, 'exp_width', 'on')
      |         set_param_state(gcb, 'frac_width', 'on')
      |     else
      |         set_param_state(gcb, 'exp_width', 'off')
      |         set_param_state(gcb, 'frac_width', 'off')
      |     end
      | 
      | 
      | else
      |     enable_fixpt = 'on'
      |     set_param_state(gcb, 'float_type', 'off')
      |     set_param_state(gcb, 'exp_width', 'off')
      |     set_param_state(gcb, 'frac_width', 'off')
      | end
      | 
      | set_param_state(gcb, 'n_bits_a', enable_fixpt)
      | set_param_state(gcb, 'bin_pt_a', enable_fixpt)
      | set_param_state(gcb, 'type_a', enable_fixpt)
      | set_param_state(gcb, 'n_bits_b', enable_fixpt)
      | set_param_state(gcb, 'bin_pt_b', enable_fixpt)
      | set_param_state(gcb, 'type_b', enable_fixpt)
      | 
      | set_param_state(gcb, 'n_bits_out', enable_fixpt)
      | set_param_state(gcb, 'bin_pt_out', enable_fixpt)
      | set_param_state(gcb, 'type_out', enable_fixpt)
      | set_param_state(gcb, 'quantization', enable_fixpt)
      | set_param_state(gcb, 'overflow', enable_fixpt)
      mask TypeOptions float_type: single | custom
      mask Callback float_type:
      | f_type = get_param(gcb, 'float_type')
      | if strcmp(f_type,'custom')
      |     set_param_state(gcb, 'exp_width', 'on')
      |     set_param_state(gcb, 'frac_width', 'on')
      | else
      |     set_param_state(gcb, 'exp_width', 'off')
      |     set_param_state(gcb, 'frac_width', 'off')
      | end
      mask TypeOptions add_implementation: behavioral HDL | fabric core | DSP48 core
  bus_register : Subsystem  mask(bus_register){reset=on, enable=off, cmplx=on, n_bits=repmat(n_bits_in, 1, 2^stream_bits), misc=on}
      mask prompts: reset "reset port"; enable "enable port"; cmplx "complex data"; n_bits "input bit widths"; misc "misc support"
      mask help: Register components of bus
      mask init:
      | bus_register_init(gcb, ...
      |     'reset', reset, ...
      |     'enable', enable, ...
      |     'cmplx', cmplx, ...
      |     'n_bits', n_bits, ...
      |     'misc', misc);
  c_to_ri : Subsystem  mask(c_to_ri){n_bits=n_bits_accum, bin_pt=bin_pt_in}
      mask prompts: n_bits "Bit Width"; bin_pt "Binary Point"
      mask help:
      | Outputs real and imaginary components of a complex input.
      | Useful for simplifying interconnects.
      | See also: Real-Imag to Complex (ri_to_c)
      mask init:
      | annotation=sprintf('%d_%d r/i',n_bits,bin_pt);
      | set_param(gcb,'AttributesFormatString',annotation);
      settings: AttributesFormatString=26_16 r/i
      mask Help: eval('xlWeb(''http://casper.berkeley.edu/wiki/C_to_ri'')')
  c_to_ri1 : Subsystem  mask(c_to_ri){n_bits=n_bits_accum, bin_pt=bin_pt_in}
      mask prompts: n_bits "Bit Width"; bin_pt "Binary Point"
      mask help:
      | Outputs real and imaginary components of a complex input.
      | Useful for simplifying interconnects.
      | See also: Real-Imag to Complex (ri_to_c)
      mask init:
      | annotation=sprintf('%d_%d r/i',n_bits,bin_pt);
      | set_param(gcb,'AttributesFormatString',annotation);
      settings: AttributesFormatString=26_16 r/i
      mask Help: eval('xlWeb(''http://casper.berkeley.edu/wiki/C_to_ri'')')
  c_to_ri2 : Subsystem  mask(c_to_ri){n_bits=n_bits_accum, bin_pt=bin_pt_in}
      mask prompts: n_bits "Bit Width"; bin_pt "Binary Point"
      mask help:
      | Outputs real and imaginary components of a complex input.
      | Useful for simplifying interconnects.
      | See also: Real-Imag to Complex (ri_to_c)
      mask init:
      | annotation=sprintf('%d_%d r/i',n_bits,bin_pt);
      | set_param(gcb,'AttributesFormatString',annotation);
      settings: AttributesFormatString=26_16 r/i
      mask Help: eval('xlWeb(''http://casper.berkeley.edu/wiki/C_to_ri'')')
  data : xbsIndex_r4/Slice  nbits=n_bits_accum*2^(stream_bits+1)  boolean_output=off  mode=Upper Bit Location + Width  bit1=0  base1=MSB of Input  bit0=0  base0=LSB of Input  dbl_ovrd=off  block_type=slice
  dump_slice : xbsIndex_r4/Slice  nbits=1  boolean_output=on  mode=Lower Bit Location + Width  bit1=0  base1=MSB of Input  bit0=2  base0=LSB of Input  dbl_ovrd=off  block_type=slice
  en_slice : xbsIndex_r4/Slice  nbits=1  boolean_output=on  mode=Lower Bit Location + Width  bit1=0  base1=MSB of Input  bit0=1  base0=LSB of Input  dbl_ovrd=off  block_type=slice
  misc : xbsIndex_r4/Slice  nbits=0  boolean_output=off  mode=Two Bit Locations  bit1=-(n_bits_accum*2^(stream_bits+1))  base1=MSB of Input  bit0=0  base0=LSB of Input  dbl_ovrd=off  block_type=slice
  misc_slice : xbsIndex_r4/Slice  nbits=1  boolean_output=off  mode=Two Bit Locations  bit1=0  base1=MSB of Input  bit0=1+1+1  base0=LSB of Input  dbl_ovrd=off  block_type=slice
  r_address : xbsIndex_r4/Counter  cnt_type=Free Running  cnt_to=Inf  operation=Up  start_count=0  cnt_by_val=1  arith_type=Unsigned  n_bits=stack_bits  bin_pt=0  load_pin=off  rst=on  en=on  explicit_period=on  period=1  use_behavioral_HDL=off  implementation=Fabric  dbl_ovrd=off  block_type=counter
      settings: block_version=11.4
  sync_slice : xbsIndex_r4/Slice  nbits=1  boolean_output=on  mode=Lower Bit Location + Width  bit1=0  base1=MSB of Input  bit0=0  base0=LSB of Input  dbl_ovrd=off  block_type=slice
  w_address : xbsIndex_r4/Counter  cnt_type=Free Running  cnt_to=Inf  operation=Up  start_count=0  cnt_by_val=1  arith_type=Unsigned  n_bits=stack_bits  bin_pt=0  load_pin=off  rst=on  en=on  explicit_period=on  period=1  use_behavioral_HDL=off  implementation=Fabric  dbl_ovrd=off  block_type=counter
      settings: block_version=11.4
  synco : Outport
  dato : Outport  Port=2
  valid : Outport  Port=3
  misc_o : Outport  Port=4
  wires:
  bus_add/2(misco) -> sync_slice/1, en_slice/1, dump_slice/1, misc_slice/1
  Gateway Out9/1 -> Scope1/8
  Gateway Out8/1 -> Scope1/7
  Gateway Out7/1 -> Scope1/6
  Gateway Out11/1 -> Scope1/5
  Gateway Out10/1 -> Scope1/4
  Gateway Out6/1 -> Scope1/3
  Gateway Out5/1 -> Scope1/2
  Gateway Out12/1 -> Scope1/1
  Gateway Out3/1 -> Scope/5
  Gateway Out2/1 -> Scope/4
  Gateway Out1/1 -> Scope/3
  Gateway Out/1 -> Scope/2
  Gateway Out4/1 -> Scope/1
  sync_slice/1 -> Delay9/1
  Delay9/1 -> Delay19/1, w_address/1, synco/1
  Delay5/1 -> Concat/4
  misc/1 -> bus_add/3(misci)
  data/1 -> bus_add/2(b)
  bus_register/2(misco) -> misc/1, data/1
  bus_register/1(dout) -> bus_add/1(a)
  Concat1/1 -> bus_register/3(misci)
  Inverter/1 -> bus_register/2(rst)
  Delay/1 -> bus_register/1(din)
  Delay2/1 -> Concat/2
  Delay4/1 -> Concat/1
  bus_add/1(dout) -> Register/1, Delay6/1
  Register/1 -> Delay12/1, acc/5
  r_address/1 -> acc/1, Delay18/1
  synci/1 -> r_address/1, Delay17/1, Delay5/1
  dat/1 -> Delay/1
  misc_in/1 -> Delay4/1
  Constant1/1 -> acc/2
  Constant2/1 -> acc/3
  misc_slice/1 -> Delay7/1
  acc/2 -> Terminator/1
  dump/1 -> Delay2/1
  Concat/1 -> Concat1/2
  acc/1 -> Delay10/1, Concat1/1
  Delay1/1 -> acc/6, Delay16/1, Delay12/2, w_address/2
  Delay3/1 -> Inverter/1
  dvalid/1 -> Delay3/1
  en/1 -> Delay8/1, r_address/2, Delay11/1
  dump_slice/1 -> Register/2, Logical/1
  en_slice/1 -> Delay1/1, Delay23/1, Logical/2
  Delay6/1 -> Delay20/1, dato/1
  Delay7/1 -> misc_o/1
  c_to_ri/1(re) -> Gateway Out/1
  c_to_ri/2(im) -> Gateway Out1/1
  c_to_ri2/1(re) -> Gateway Out6/1
  c_to_ri2/2(im) -> Gateway Out10/1
  c_to_ri1/1(re) -> Gateway Out7/1
  c_to_ri1/2(im) -> Gateway Out8/1
  Logical/1 -> valid/1, Delay21/1, Delay20/2
  Delay8/1 -> Concat/3
  Delay10/1 -> c_to_ri2/1(c)
  Delay11/1 -> Delay10/2
  w_address/1 -> Delay15/1, acc/4
  Delay13/1 -> Gateway Out12/1
  Delay14/1 -> Gateway Out5/1
  Delay15/1 -> Gateway Out11/1
  Delay16/1 -> Gateway Out9/1
  Delay12/1 -> c_to_ri1/1(c)
  Delay17/1 -> Delay13/1
  Delay18/1 -> Delay14/1
  Delay20/1 -> c_to_ri/1(c)
  Delay19/1 -> Gateway Out4/1
  Delay21/1 -> Gateway Out2/1
  Delay22/1 -> Gateway Out3/1
  Delay23/1 -> Delay22/1
